simulink model "BEVModel_WLTP"  (R2023b)
settings: Solver=VariableStepAuto  StartTime=0.0  StopTime=1800  RelTol=1e-3
values from neighbouring files (symbols this model uses):
  Aero_F = 0.5 * cw * A * rho * rdyn^2    (= 0.04094064)    [Parameters.m]
  dm = 7    [Parameters.m]
  dr = 196    [Parameters.m]
  Fa = (mr + Vm)*rdyn    (= 449.8672189)    [Parameters.m]
  i_total = 10.1    [Parameters.m]
  Imot = 1    [Parameters.m]
  Ir = Vm * rdyn^2 / i_total^2    (= 1.17914910303)    [Parameters.m]
  Itrans = 1.2    [Parameters.m]
  km = 10000    [Parameters.m]
  kr = 191.5    [Parameters.m]
  rdyn = 0.27    [Parameters.m]
  Roll_F = fr * Vm * g    (= 275.1705)    [Parameters.m]
  T = [T1 T1 T2 T3 0]'    [Parameters.m]
  W = [0 W1 W2 W3 W3+5]'    [Parameters.m]
libraries: simulink x1, slpidlib x1
settings Model: Creator=dinul  LastModifiedBy=dinul
settings DataIOCC: ReturnWorkspaceOutputs=off
settings DebuggingCC: AlgebraicLoopMsg=none  ArtificialAlgebraicLoopMsg=none  OperatingPointInterfaceChecksumMismatchMsg=none

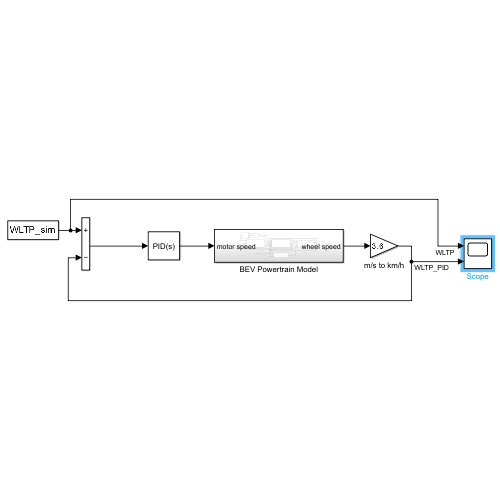
[thumbnail: Simulink's stored preview of the top-level diagram]
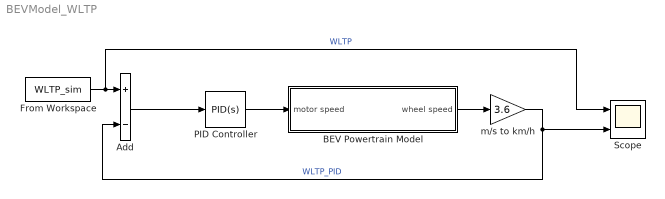
== system BEVModel_WLTP ==
  Add : Sum  Inputs=+-
  BEV Powertrain Model : Subsystem
  From Workspace : FromWorkspace  VariableName=WLTP_sim
  PID Controller : slpidlib/PID Controller  Controller=PID  Form=Parallel  TimeDomain=Continuous-time  UseExternalTs=off  SampleTime=-1  IntegratorMethod=Forward Euler  FilterMethod=Forward Euler  ControllerParametersSource=internal  P=50  I=0  UseKiTs=off  D=7  N=100  UseFilter=on  TunerSelectOption=Transfer Function Based (PID Tuner App)  InitialConditionSource=internal  InitialConditionForIntegrator=0  InitialConditionForFilter=0  DifferentiatorICPrevScaledInput=0  ExternalReset=none  TrackingMode=off  Kt=1  LimitOutput=off  SatLimitsSource=internal  UpperSaturationLimit=inf  LowerSaturationLimit=-inf  LinearizeAsGain=on  AntiWindupMode=none  Kb=1  LimitIntegrator=off  UpperIntegratorSaturationLimit=inf  LowerIntegratorSaturationLimit=-inf  POutMin=[]  POutMax=[]  IOutMin=[]  IOutMax=[]  DOutMin=[]  DOutMax=[]  NOutMin=[]  NOutMax=[]  SumOutMin=[]  SumOutMax=[]  SaturationOutMin=[]  SaturationOutMax=[]  PParamMin=[]  PParamMax=[]  IParamMin=[]  IParamMax=[]  DParamMin=[]  DParamMax=[]  NParamMin=[]  NParamMax=[]  KbParamMin=[]  KbParamMax=[]  KtParamMin=[]  KtParamMax=[]  KbOutMin=[]  KbOutMax=[]  KtOutMin=[]  KtOutMax=[]  IntegratorOutMin=[]  IntegratorOutMax=[]  FilterOutMin=[]  FilterOutMax=[]  SumI1OutMin=[]  SumI1OutMax=[]  SumI2OutMin=[]  SumI2OutMax=[]  SumI3OutMin=[]  SumI3OutMax=[]  SumI4OutMin=[]  SumI4OutMax=[]  SumDOutMin=[]  SumDOutMax=[]  DifferentiatorOutMin=[]  DifferentiatorOutMax=[]  FilterDiffOutCoefMin=[]  FilterDiffOutCoefMax=[]  ReciprocalOutMin=[]  ReciprocalOutMax=[]  SumDenOutMin=[]  SumDenOutMax=[]  SumNumOutMin=[]  SumNumOutMax=[]  DivideOutMin=[]  DivideOutMax=[]  UdiffTsProdOutMin=[]  UdiffTsProdOutMax=[]  NTsProdOutMin=[]  NTsProdOutMax=[]  UintegralTsProdOutMin=[]  UintegralTsProdOutMax=[]  UngainTsProdOutMin=[]  UngainTsProdOutMax=[]  ClampingZeroOutDataTypeStr=Inherit: Inherit via back propagation  ClampingZeroOutMin=[]  ClampingZeroOutMax=[]  FilterDenConstantOutDataTypeStr=Inherit: Inherit via back propagation  FilterDenConstantOutMin=[]  FilterDenConstantOutMax=[]  PCopyOutDataTypeStr=Inherit: Inherit via back propagation  PCopyOutMin=[]  PCopyOutMax=[]  NCopyOutDataTypeStr=Inherit: Inherit via back propagation  NCopyOutMin=[]  NCopyOutMax=[]  IntegratorContinuousStateAttributes=''  IntegratorStateMustResolveToSignalObject=off  IntegratorRTWStateStorageClass=Auto  FilterContinuousStateAttributes=''  FilterStateMustResolveToSignalObject=off  FilterRTWStateStorageClass=Auto  ParallelPVariant=InternalParameters  IdealPVariant=Disabled  IVariant=InternalParameters  DVariant=InternalParameters  IntegratorVariant=Continuous  SatVariant=Disabled  AWVariant=Passthrough  PCopyVariant=Disabled  TRVariant=Disabled  FdbkBlocksVariant=Forward  IdealPFdbkVariant=Disabled  SatFdbkVariant=Disabled  DerivativeFilterVariant=ContFilter  NVariant=InternalParameters  NCopyVariant=Disabled  FilterICVariant=InternalICsFilter  IntegratorICVariant=InternalICs  ExternalResetVariant=Disabled  TRSumVariant=Passthrough  SumFdbkVariant=Disabled  SumVariant=Sum_PID  TsampFilterVariant=InternalTs  TsampNgainVariant=Passthrough  TsampIntegralVariant=Disabled_SignalSpec  ExternalSaturationOutDataTypeStr=Inherit: Same as second input
  Scope : Scope  NumInputPorts=2
  m/s to km/h : Gain  Gain=3.6
  wires:
  From Workspace/1 -> Scope/1, Add/1  "WLTP"
  Add/1 -> PID Controller/1
  m/s to km/h/1 -> Scope/2, Add/2  "WLTP_PID"
  PID Controller/1 -> BEV Powertrain Model/1(motor speed)
  BEV Powertrain Model/1(wheel speed) -> m/s to km/h/1

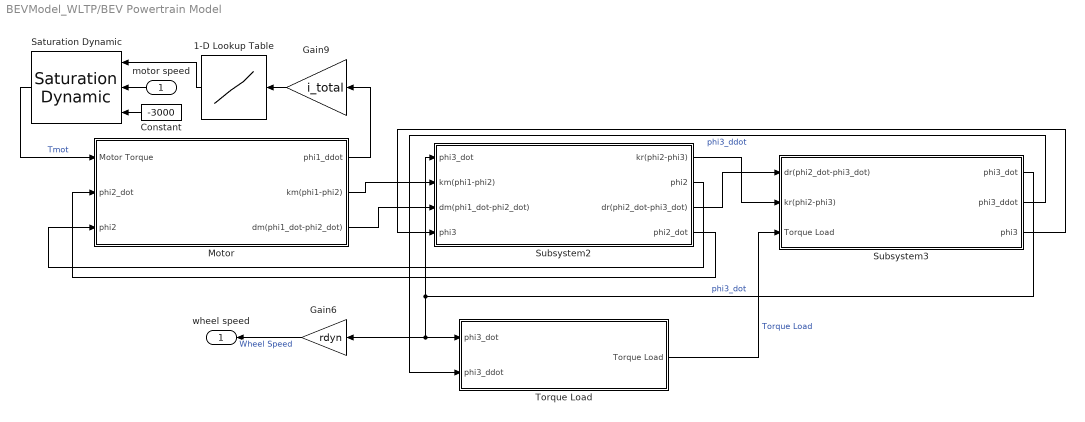
== system BEVModel_WLTP/BEV Powertrain Model ==
  motor speed : Inport
  1-D Lookup Table : Lookup_n-D  NumberOfTableDimensions=1  BreakpointsForDimension1=W  Table=T  InternalRulePriority=Speed  RndMeth=Simplest
  Constant : Constant  Value=-3000
  Gain6 : Gain  Gain=rdyn
  Gain9 : Gain  Gain=i_total
  Motor : Subsystem
  Saturation Dynamic : simulink/Discontinuities/Saturation Dynamic  OutMin=[]  OutMax=[]  OutDataTypeStr=Inherit: Inherit via back propagation  OutDataType=fixdt(1, 16)  OutScaling=2^-10  DoSatur=off
  Subsystem2 : Subsystem
  Subsystem3 : Subsystem
  Torque Load : Subsystem
  wheel speed : Outport
  wires:
  Gain6/1 -> wheel speed/1  "Wheel Speed"
  Gain9/1 -> 1-D Lookup Table/1
  motor speed/1 -> Saturation Dynamic/2
  1-D Lookup Table/1 -> Saturation Dynamic/1
  Constant/1 -> Saturation Dynamic/3
  Saturation Dynamic/1 -> Motor/1(Motor Torque)  "Tmot"
  Torque Load/1(Torque Load) -> Subsystem3/3(Torque Load)  "Torque Load"
  Subsystem3/1(phi3_dot) -> Subsystem2/1(phi3_dot), Gain6/1, Torque Load/1(phi3_dot)  "phi3_dot"
  Subsystem3/2(phi3_ddot) -> Torque Load/2(phi3_ddot)  "phi3_ddot"
  Subsystem2/4(phi2_dot) -> Motor/2(phi2_dot)
  Motor/2(km(phi1-phi2)) -> Subsystem2/2(km(phi1-phi2))
  Subsystem2/2(phi2) -> Motor/3(phi2)
  Subsystem2/3(dr(phi2_dot-phi3_dot)) -> Subsystem3/1(dr(phi2_dot-phi3_dot))
  Subsystem2/1(kr(phi2-phi3)) -> Subsystem3/2(kr(phi2-phi3))
  Subsystem3/3(phi3) -> Subsystem2/4(phi3)
  Motor/3(dm(phi1_dot-phi2_dot)) -> Subsystem2/3(dm(phi1_dot-phi2_dot))
  Motor/1(phi1_ddot) -> Gain9/1

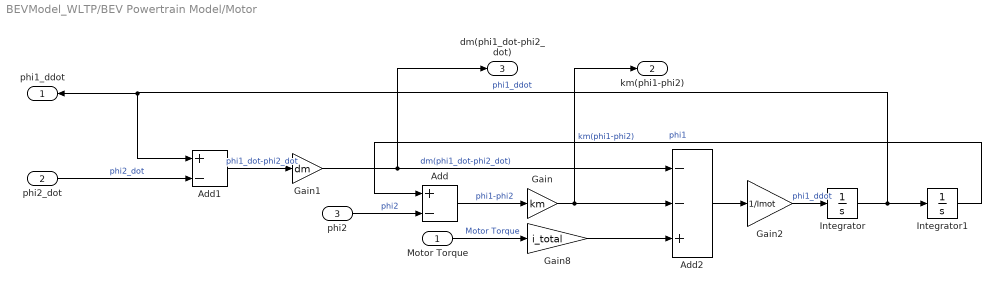
== system BEVModel_WLTP/BEV Powertrain Model/Motor ==
  Motor Torque : Inport
  phi2_dot : Inport  Port=2
  phi2 : Inport  Port=3
  Add : Sum  Inputs=+-
  Add1 : Sum  Inputs=+-
  Add2 : Sum  Inputs=--+
  Gain : Gain  Gain=km
  Gain1 : Gain  Gain=dm
  Gain2 : Gain  Gain=1/Imot
  Gain8 : Gain  Gain=i_total
  Integrator : Integrator
  Integrator1 : Integrator
  phi1_ddot : Outport
  km(phi1-phi2) : Outport  Port=2
  dm(phi1_dot-phi2_dot) : Outport  Port=3
  wires:
  Gain/1 -> km(phi1-phi2)/1, Add2/2  "km(phi1-phi2)"
  Add2/1 -> Gain2/1
  Add1/1 -> Gain1/1  "phi1_dot-phi2_dot"
  Add/1 -> Gain/1  "phi1-phi2"
  Integrator/1 -> phi1_ddot/1, Add1/1, Integrator1/1  "phi1_ddot"
  Integrator1/1 -> Add/1  "phi1"
  Gain1/1 -> dm(phi1_dot-phi2_dot)/1, Add2/1  "dm(phi1_dot-phi2_dot)"
  phi2/1 -> Add/2  "phi2"
  Gain2/1 -> Integrator/1  "phi1_ddot"
  phi2_dot/1 -> Add1/2  "phi2_dot"
  Gain8/1 -> Add2/3
  Motor Torque/1 -> Gain8/1  "Motor Torque"

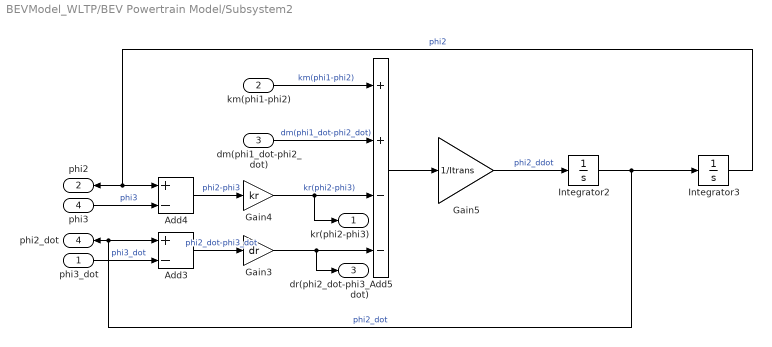
== system BEVModel_WLTP/BEV Powertrain Model/Subsystem2 ==
  phi3_dot : Inport
  km(phi1-phi2) : Inport  Port=2
  dm(phi1_dot-phi2_dot) : Inport  Port=3
  phi3 : Inport  Port=4
  Add3 : Sum  Inputs=+-
  Add4 : Sum  Inputs=+-
  Add5 : Sum  Inputs=++--
  Gain3 : Gain  Gain=dr
  Gain4 : Gain  Gain=kr
  Gain5 : Gain  Gain=1/Itrans
  Integrator2 : Integrator
  Integrator3 : Integrator
  kr(phi2-phi3) : Outport
  phi2 : Outport  Port=2
  dr(phi2_dot-phi3_dot) : Outport  Port=3
  phi2_dot : Outport  Port=4
  wires:
  km(phi1-phi2)/1 -> Add5/1  "km(phi1-phi2)"
  Gain3/1 -> dr(phi2_dot-phi3_dot)/1, Add5/4
  Integrator2/1 -> Integrator3/1, Add3/1, phi2_dot/1  "phi2_dot"
  Integrator3/1 -> phi2/1, Add4/1  "phi2"
  Add5/1 -> Gain5/1
  phi3_dot/1 -> Add3/2  "phi3_dot"
  Add3/1 -> Gain3/1  "phi2_dot-phi3_dot"
  phi3/1 -> Add4/2  "phi3"
  Gain5/1 -> Integrator2/1  "phi2_ddot"
  Gain4/1 -> kr(phi2-phi3)/1, Add5/3  "kr(phi2-phi3)"
  dm(phi1_dot-phi2_dot)/1 -> Add5/2  "dm(phi1_dot-phi2_dot)"
  Add4/1 -> Gain4/1  "phi2-phi3"

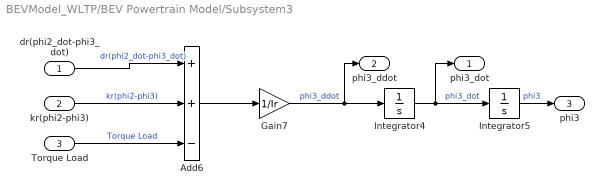
== system BEVModel_WLTP/BEV Powertrain Model/Subsystem3 ==
  dr(phi2_dot-phi3_dot) : Inport
  kr(phi2-phi3) : Inport  Port=2
  Torque Load : Inport  Port=3
  Add6 : Sum  Inputs=++-
  Gain7 : Gain  Gain=1/Ir
  Integrator4 : Integrator
  Integrator5 : Integrator
  phi3_dot : Outport
  phi3_ddot : Outport  Port=2
  phi3 : Outport  Port=3
  wires:
  kr(phi2-phi3)/1 -> Add6/2  "kr(phi2-phi3)"
  Integrator5/1 -> phi3/1  "phi3"
  Torque Load/1 -> Add6/3  "Torque Load"
  Gain7/1 -> phi3_ddot/1, Integrator4/1  "phi3_ddot"
  Add6/1 -> Gain7/1
  dr(phi2_dot-phi3_dot)/1 -> Add6/1  "dr(phi2_dot-phi3_dot)"
  Integrator4/1 -> phi3_dot/1, Integrator5/1  "phi3_dot"

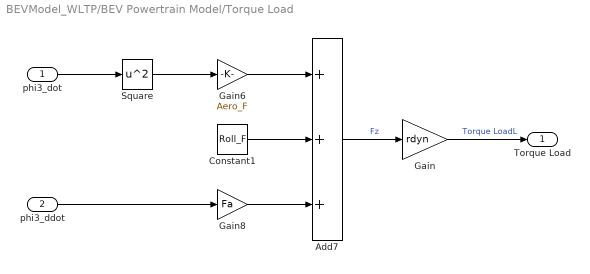
== system BEVModel_WLTP/BEV Powertrain Model/Torque Load ==
  phi3_dot : Inport
  phi3_ddot : Inport  Port=2
  Add7 : Sum  Inputs=+++
  Constant1 : Constant  Value=Roll_F
  Gain : Gain  Gain=rdyn
  Gain6 : Gain  Gain=Aero_F
  Gain8 : Gain  Gain=Fa
  Square : Math  Operator=square
  Torque Load : Outport
  wires:
  Square/1 -> Gain6/1
  Gain8/1 -> Add7/3
  phi3_dot/1 -> Square/1
  Gain6/1 -> Add7/1
  phi3_ddot/1 -> Gain8/1
  Constant1/1 -> Add7/2
  Add7/1 -> Gain/1  "Fz"
  Gain/1 -> Torque Load/1  "Torque LoadL"
